simulink model "Sincronizador_model"  (Simulink 8.8)
settings: Solver=ode113  StartTime=0.0  StopTime=10  FixedStep=0.0000000001  RelTol=1e-8  EnableMultiTasking=on
settings Model: Creator=kevinhmg  LastModifiedBy=Kevinhmg
settings DataIOCC: LimitDataPoints=off  TimeSaveName=t
settings OptimizationCC: ExpressionDepthLimit=2147483647
settings DebuggingCC: SolverPrmCheckMsg=warning

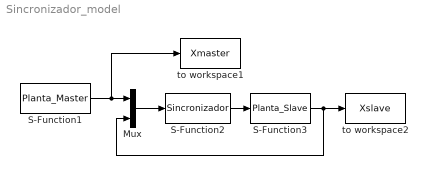
== system Sincronizador_model ==
  Mux : Mux  Inputs=2
  S-Function1 : S-Function  FunctionName=Planta_Master  SFunctionDeploymentMode=off  EnableBusSupport=off
  S-Function2 : S-Function  FunctionName=Sincronizador  SFunctionDeploymentMode=off  EnableBusSupport=off
  S-Function3 : S-Function  FunctionName=Planta_Slave  SFunctionDeploymentMode=off  EnableBusSupport=off
  to workspace1 : ToWorkspace  VariableName=Xmaster  SampleTime=-1
  to workspace2 : ToWorkspace  VariableName=Xslave  SampleTime=-1
  wires:
  S-Function2/1 -> S-Function3/1
  S-Function3/1 -> to workspace2/1, Mux/2
  S-Function1/1 -> to workspace1/1, Mux/1
  Mux/1 -> S-Function2/1
